simulink library "G474_Firmware_PI"  (R2024b)
settings: Solver=VariableStepAuto  StartTime=0.0  StopTime=10.0  RelTol=1e-3
settings Model: Creator=QXZ-030079  LastModifiedBy=QXZ-030079

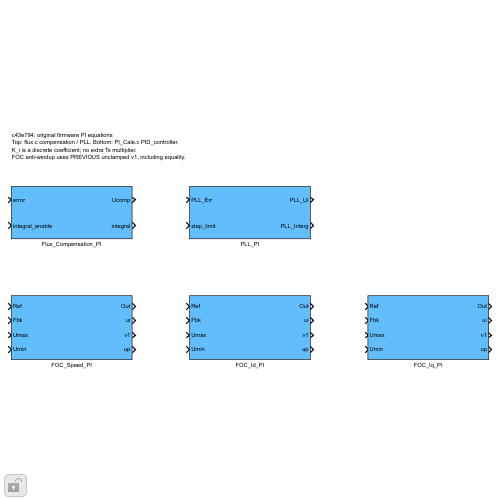
[thumbnail: Simulink's stored preview of the top-level diagram]
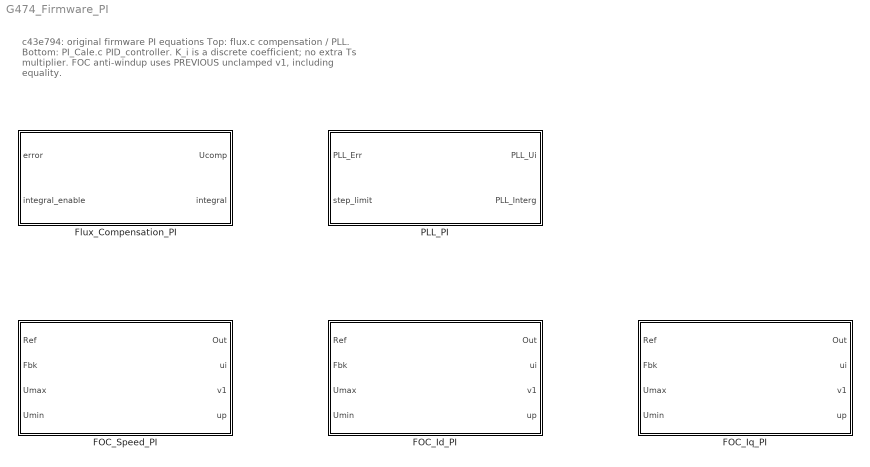
== system G474_Firmware_PI ==
  note: c43e794: original firmware PI equations
      | Top: flux.c compensation / PLL. Bottom: PI_Cale.c PID_controller.
      | K_i is a discrete coefficient; no extra Ts multiplier.
      | FOC anti-windup uses PREVIOUS unclamped v1, including equality.
  FOC_Id_PI : Subsystem  mask{Kp=0.01, Ki=0.00001, Ts=5e-5}
      mask prompts: Kp "Kp (source coefficient)"; Ki "Ki (per call, already discrete)"; Ts "Execution period (s)"
      settings: OpenFcn=open_system(gcb,'force')
      mask Display: port_label('input',1,'Ref');port_label('input',2,'Fbk');port_label('input',3,'Umax');port_label('input',4,'Umin');port_label('output',1,'Out');port_label('output',2,'ui');port_label('output',3,'v1');port_label('output',4,'up');
  FOC_Iq_PI : Subsystem  mask{Kp=0.01, Ki=0.00001, Ts=5e-5}
      mask prompts: Kp "Kp (source coefficient)"; Ki "Ki (per call, already discrete)"; Ts "Execution period (s)"
      settings: OpenFcn=open_system(gcb,'force')
      mask Display: port_label('input',1,'Ref');port_label('input',2,'Fbk');port_label('input',3,'Umax');port_label('input',4,'Umin');port_label('output',1,'Out');port_label('output',2,'ui');port_label('output',3,'v1');port_label('output',4,'up');
  FOC_Speed_PI : Subsystem  mask{Kp=0.01, Ki=0.0001, Ts=5e-5}
      mask prompts: Kp "Kp (source coefficient)"; Ki "Ki (per call, already discrete)"; Ts "Execution period (s)"
      settings: OpenFcn=open_system(gcb,'force')
      mask Display: port_label('input',1,'Ref');port_label('input',2,'Fbk');port_label('input',3,'Umax');port_label('input',4,'Umin');port_label('output',1,'Out');port_label('output',2,'ui');port_label('output',3,'v1');port_label('output',4,'up');
  Flux_Compensation_PI : Subsystem  mask{Kp=62.831853071795862, Ki=0.049348022005446794, Ts=5e-5}
      mask prompts: Kp "Kp (source coefficient)"; Ki "Ki (per call, already discrete)"; Ts "Execution period (s)"
      settings: OpenFcn=open_system(gcb,'force')
      mask Display: port_label('input',1,'error');port_label('input',2,'integral_enable');port_label('output',1,'Ucomp');port_label('output',2,'integral');
  PLL_PI : Subsystem  mask{Kp=188.49555921538757, Ki=0.44413219804902104, Ts=5e-5}
      mask prompts: Kp "Kp (source coefficient)"; Ki "Ki (per call, already discrete)"; Ts "Execution period (s)"
      settings: OpenFcn=open_system(gcb,'force')
      mask Display: port_label('input',1,'PLL_Err');port_label('input',2,'step_limit');port_label('output',1,'PLL_Ui');port_label('output',2,'PLL_Interg');

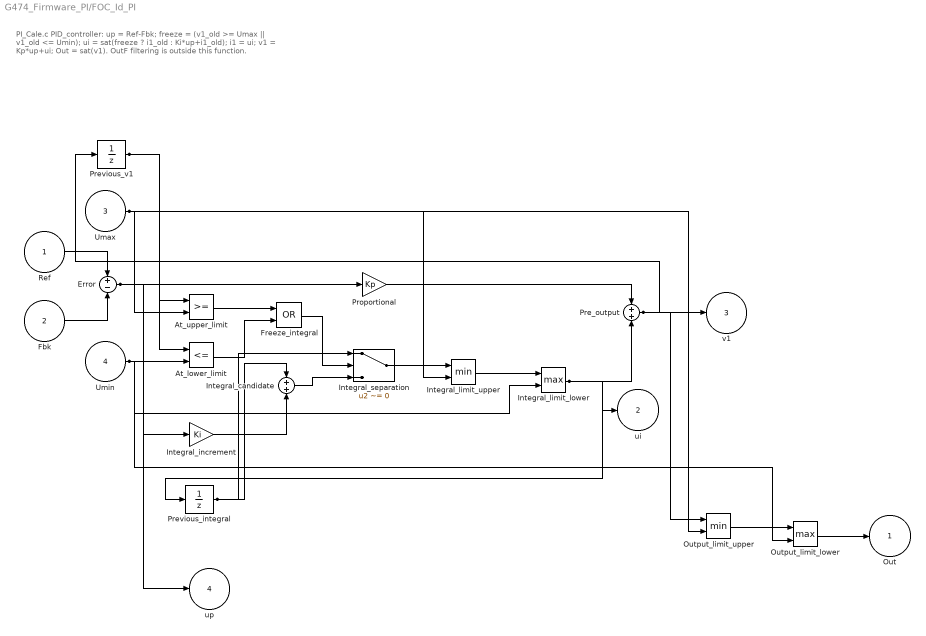
== system G474_Firmware_PI/FOC_Id_PI ==
  note: PI_Cale.c PID_controller:
      | up = Ref-Fbk; freeze = (v1_old >= Umax || v1_old <= Umin);
      | ui = sat(freeze ? i1_old : Ki*up+i1_old); i1 = ui;
      | v1 = Kp*up+ui; Out = sat(v1). OutF filtering is outside this function.
  Ref : Inport
  Fbk : Inport  Port=2
  Umax : Inport  Port=3
  Umin : Inport  Port=4
  At_lower_limit : RelationalOperator  Operator=<=  OutDataTypeStr=boolean  RndMeth=Simplest  InputSameDT=off
  At_upper_limit : RelationalOperator  OutDataTypeStr=boolean  RndMeth=Simplest  InputSameDT=off
  Error : Sum  Inputs=+-
  Freeze_integral : Logic  Operator=OR  AllPortsSameDT=off  OutDataTypeStr=boolean
  Integral_candidate : Sum
  Integral_increment : Gain  Gain=Ki
  Integral_limit_lower : MinMax  Function=max  Inputs=2
  Integral_limit_upper : MinMax  Inputs=2
  Integral_separation : Switch  Criteria=u2 ~= 0  SaturateOnIntegerOverflow=off  InputSameDT=off
  Output_limit_lower : MinMax  Function=max  Inputs=2
  Output_limit_upper : MinMax  Inputs=2
  Pre_output : Sum
  Previous_integral : UnitDelay  SampleTime=Ts  HasFrameUpgradeWarning=on
  Previous_v1 : UnitDelay  SampleTime=Ts  HasFrameUpgradeWarning=on
  Proportional : Gain  Gain=Kp
  Out : Outport
  ui : Outport  Port=2
  v1 : Outport  Port=3
  up : Outport  Port=4
  wires:
  At_lower_limit/1 -> Freeze_integral/2
  Ref/1 -> Error/1
  Umin/1 -> Integral_limit_lower/2, Output_limit_lower/2, At_lower_limit/2
  Fbk/1 -> Error/2
  Umax/1 -> Integral_limit_upper/2, Output_limit_upper/2, At_upper_limit/2
  Previous_v1/1 -> At_upper_limit/1, At_lower_limit/1
  Error/1 -> Proportional/1, up/1, Integral_increment/1
  At_upper_limit/1 -> Freeze_integral/1
  Integral_increment/1 -> Integral_candidate/2
  Previous_integral/1 -> Integral_candidate/1, Integral_separation/1
  Freeze_integral/1 -> Integral_separation/2
  Integral_candidate/1 -> Integral_separation/3
  Proportional/1 -> Pre_output/1
  Integral_separation/1 -> Integral_limit_upper/1
  Integral_limit_upper/1 -> Integral_limit_lower/1
  Integral_limit_lower/1 -> Pre_output/2, ui/1, Previous_integral/1
  Pre_output/1 -> Previous_v1/1, v1/1, Output_limit_upper/1
  Output_limit_upper/1 -> Output_limit_lower/1
  Output_limit_lower/1 -> Out/1

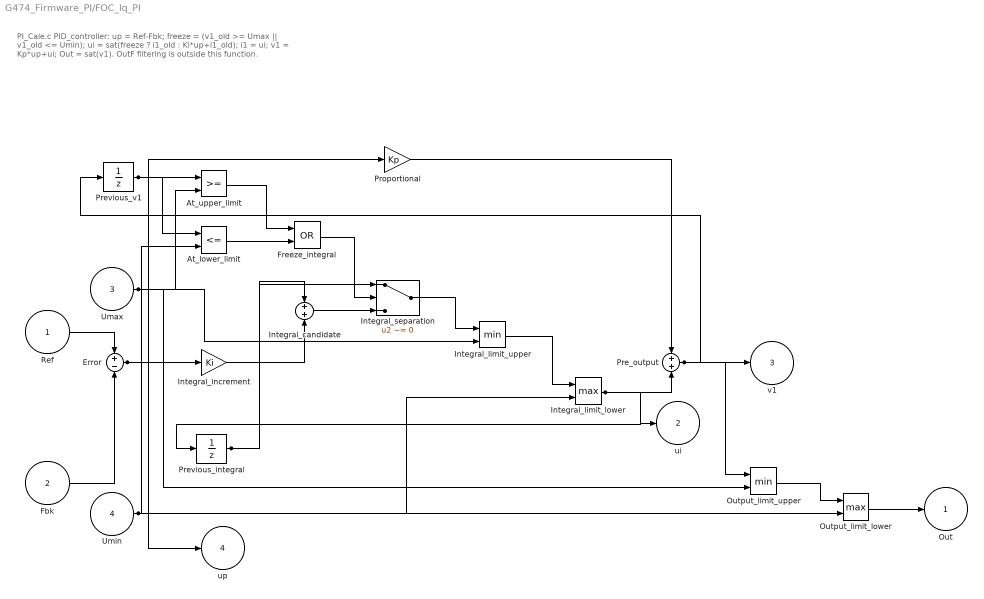
== system G474_Firmware_PI/FOC_Iq_PI ==
  note: PI_Cale.c PID_controller:
      | up = Ref-Fbk; freeze = (v1_old >= Umax || v1_old <= Umin);
      | ui = sat(freeze ? i1_old : Ki*up+i1_old); i1 = ui;
      | v1 = Kp*up+ui; Out = sat(v1). OutF filtering is outside this function.
  Ref : Inport
  Fbk : Inport  Port=2
  Umax : Inport  Port=3
  Umin : Inport  Port=4
  At_lower_limit : RelationalOperator  Operator=<=  OutDataTypeStr=boolean  RndMeth=Simplest  InputSameDT=off
  At_upper_limit : RelationalOperator  OutDataTypeStr=boolean  RndMeth=Simplest  InputSameDT=off
  Error : Sum  Inputs=+-
  Freeze_integral : Logic  Operator=OR  AllPortsSameDT=off  OutDataTypeStr=boolean
  Integral_candidate : Sum
  Integral_increment : Gain  Gain=Ki
  Integral_limit_lower : MinMax  Function=max  Inputs=2
  Integral_limit_upper : MinMax  Inputs=2
  Integral_separation : Switch  Criteria=u2 ~= 0  SaturateOnIntegerOverflow=off  InputSameDT=off
  Output_limit_lower : MinMax  Function=max  Inputs=2
  Output_limit_upper : MinMax  Inputs=2
  Pre_output : Sum
  Previous_integral : UnitDelay  SampleTime=Ts  HasFrameUpgradeWarning=on
  Previous_v1 : UnitDelay  SampleTime=Ts  HasFrameUpgradeWarning=on
  Proportional : Gain  Gain=Kp
  Out : Outport
  ui : Outport  Port=2
  v1 : Outport  Port=3
  up : Outport  Port=4
  wires:
  At_lower_limit/1 -> Freeze_integral/2
  Ref/1 -> Error/1
  Umin/1 -> Integral_limit_lower/2, At_lower_limit/2, Output_limit_lower/2
  Fbk/1 -> Error/2
  Umax/1 -> Integral_limit_upper/2, Output_limit_upper/2, At_upper_limit/2
  Previous_v1/1 -> At_upper_limit/1, At_lower_limit/1
  At_upper_limit/1 -> Freeze_integral/1
  Error/1 -> Proportional/1, up/1, Integral_increment/1
  Integral_increment/1 -> Integral_candidate/2
  Previous_integral/1 -> Integral_candidate/1, Integral_separation/1
  Output_limit_lower/1 -> Out/1
  Freeze_integral/1 -> Integral_separation/2
  Integral_candidate/1 -> Integral_separation/3
  Proportional/1 -> Pre_output/1
  Integral_separation/1 -> Integral_limit_upper/1
  Integral_limit_upper/1 -> Integral_limit_lower/1
  Integral_limit_lower/1 -> Previous_integral/1, Pre_output/2, ui/1
  Pre_output/1 -> v1/1, Previous_v1/1, Output_limit_upper/1
  Output_limit_upper/1 -> Output_limit_lower/1

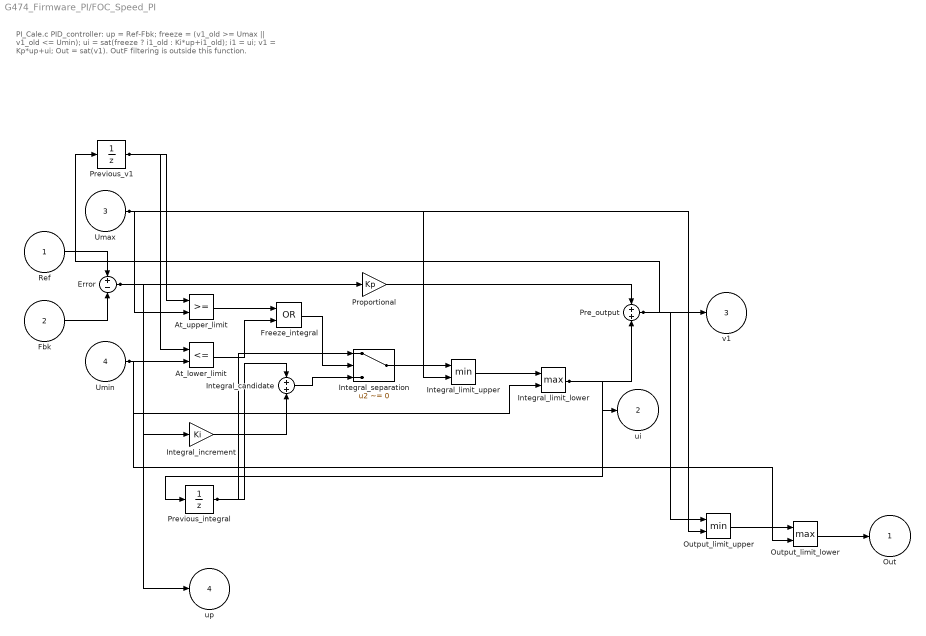
== system G474_Firmware_PI/FOC_Speed_PI ==
  note: PI_Cale.c PID_controller:
      | up = Ref-Fbk; freeze = (v1_old >= Umax || v1_old <= Umin);
      | ui = sat(freeze ? i1_old : Ki*up+i1_old); i1 = ui;
      | v1 = Kp*up+ui; Out = sat(v1). OutF filtering is outside this function.
  Ref : Inport
  Fbk : Inport  Port=2
  Umax : Inport  Port=3
  Umin : Inport  Port=4
  At_lower_limit : RelationalOperator  Operator=<=  OutDataTypeStr=boolean  RndMeth=Simplest  InputSameDT=off
  At_upper_limit : RelationalOperator  OutDataTypeStr=boolean  RndMeth=Simplest  InputSameDT=off
  Error : Sum  Inputs=+-
  Freeze_integral : Logic  Operator=OR  AllPortsSameDT=off  OutDataTypeStr=boolean
  Integral_candidate : Sum
  Integral_increment : Gain  Gain=Ki
  Integral_limit_lower : MinMax  Function=max  Inputs=2
  Integral_limit_upper : MinMax  Inputs=2
  Integral_separation : Switch  Criteria=u2 ~= 0  SaturateOnIntegerOverflow=off  InputSameDT=off
  Output_limit_lower : MinMax  Function=max  Inputs=2
  Output_limit_upper : MinMax  Inputs=2
  Pre_output : Sum
  Previous_integral : UnitDelay  SampleTime=Ts  HasFrameUpgradeWarning=on
  Previous_v1 : UnitDelay  SampleTime=Ts  HasFrameUpgradeWarning=on
  Proportional : Gain  Gain=Kp
  Out : Outport
  ui : Outport  Port=2
  v1 : Outport  Port=3
  up : Outport  Port=4
  wires:
  At_lower_limit/1 -> Freeze_integral/2
  Integral_limit_lower/1 -> Previous_integral/1, Pre_output/2, ui/1
  Ref/1 -> Error/1
  Integral_separation/1 -> Integral_limit_upper/1
  Fbk/1 -> Error/2
  Previous_v1/1 -> At_lower_limit/1, At_upper_limit/1
  Previous_integral/1 -> Integral_candidate/1, Integral_separation/1
  Umax/1 -> Integral_limit_upper/2, Output_limit_upper/2, At_upper_limit/2
  Error/1 -> Proportional/1, up/1, Integral_increment/1
  At_upper_limit/1 -> Freeze_integral/1
  Umin/1 -> Output_limit_lower/2, Integral_limit_lower/2, At_lower_limit/2
  Integral_increment/1 -> Integral_candidate/2
  Freeze_integral/1 -> Integral_separation/2
  Output_limit_upper/1 -> Output_limit_lower/1
  Integral_candidate/1 -> Integral_separation/3
  Proportional/1 -> Pre_output/1
  Integral_limit_upper/1 -> Integral_limit_lower/1
  Pre_output/1 -> Previous_v1/1, v1/1, Output_limit_upper/1
  Output_limit_lower/1 -> Out/1

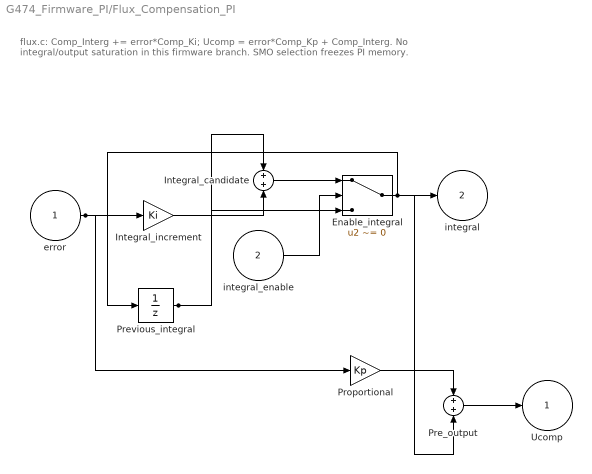
== system G474_Firmware_PI/Flux_Compensation_PI ==
  note: flux.c: Comp_Interg += error*Comp_Ki; Ucomp = error*Comp_Kp + Comp_Interg.
      | No integral/output saturation in this firmware branch. SMO selection freezes PI memory.
  error : Inport
  integral_enable : Inport  Port=2
  Enable_integral : Switch  Criteria=u2 ~= 0  SaturateOnIntegerOverflow=off  InputSameDT=off
  Integral_candidate : Sum
  Integral_increment : Gain  Gain=Ki
  Pre_output : Sum
  Previous_integral : UnitDelay  SampleTime=Ts  HasFrameUpgradeWarning=on
  Proportional : Gain  Gain=Kp
  Ucomp : Outport
  integral : Outport  Port=2
  wires:
  error/1 -> Proportional/1, Integral_increment/1
  Enable_integral/1 -> Pre_output/2, integral/1, Previous_integral/1
  Integral_increment/1 -> Integral_candidate/2
  Previous_integral/1 -> Enable_integral/3, Integral_candidate/1
  Integral_candidate/1 -> Enable_integral/1
  integral_enable/1 -> Enable_integral/2
  Proportional/1 -> Pre_output/1
  Pre_output/1 -> Ucomp/1

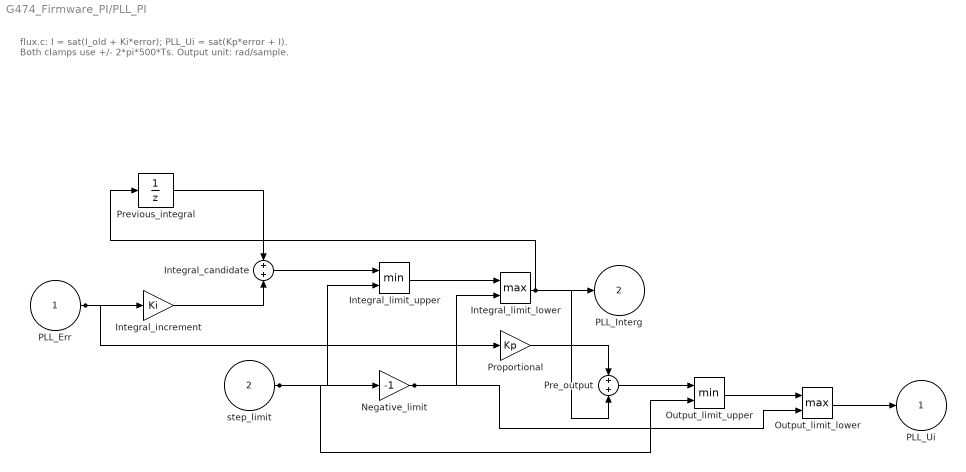
== system G474_Firmware_PI/PLL_PI ==
  note: flux.c: I = sat(I_old + Ki*error); PLL_Ui = sat(Kp*error + I).
      | Both clamps use +/- 2*pi*500*Ts. Output unit: rad/sample.
  PLL_Err : Inport
  step_limit : Inport  Port=2
  Integral_candidate : Sum
  Integral_increment : Gain  Gain=Ki
  Integral_limit_lower : MinMax  Function=max  Inputs=2
  Integral_limit_upper : MinMax  Inputs=2
  Negative_limit : Gain  Gain=-1
  Output_limit_lower : MinMax  Function=max  Inputs=2
  Output_limit_upper : MinMax  Inputs=2
  Pre_output : Sum
  Previous_integral : UnitDelay  SampleTime=Ts  HasFrameUpgradeWarning=on
  Proportional : Gain  Gain=Kp
  PLL_Ui : Outport
  PLL_Interg : Outport  Port=2
  wires:
  PLL_Err/1 -> Integral_increment/1, Proportional/1
  step_limit/1 -> Output_limit_upper/2, Negative_limit/1, Integral_limit_upper/2
  Previous_integral/1 -> Integral_candidate/1
  Integral_increment/1 -> Integral_candidate/2
  Integral_limit_lower/1 -> Pre_output/2, PLL_Interg/1, Previous_integral/1
  Integral_candidate/1 -> Integral_limit_upper/1
  Integral_limit_upper/1 -> Integral_limit_lower/1
  Negative_limit/1 -> Output_limit_lower/2, Integral_limit_lower/2
  Proportional/1 -> Pre_output/1
  Pre_output/1 -> Output_limit_upper/1
  Output_limit_upper/1 -> Output_limit_lower/1
  Output_limit_lower/1 -> PLL_Ui/1
